simulink model "part1_pendulum_R2021a"  (R2021a)
settings: Solver=ode45  StartTime=0.0  StopTime=2  MaxStep=0.005  RelTol=1e-8  AbsTol=1e-10
model workspace (MAT data in the model file):
  g = 9.81
  k = 0.05
  l = 0.5
  m = 0.2
  omega0 = 0
  theta0 = 0.1
settings Model: Creator=matiasgarcia  LastModifiedBy=matiasgarcia
settings DataIOCC: SaveOutput=off  SignalLogging=off  SaveTime=off
settings DebuggingCC: UnconnectedInputMsg=none  UnconnectedOutputMsg=none  UnconnectedLineMsg=none
settings ModelReferenceCC: EnableRefExpFcnMdlSchedulingChecks=off
settings RTWCC: Description=Generic Real-Time Target  GPUComputeCapability=5.0  DLArmComputeVersion=20.02.1

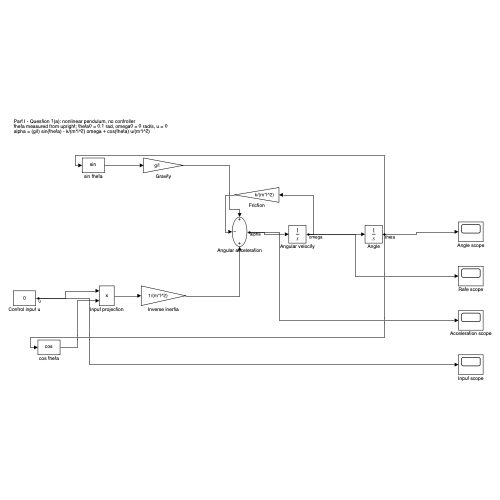
[thumbnail: Simulink's stored preview of the top-level diagram]
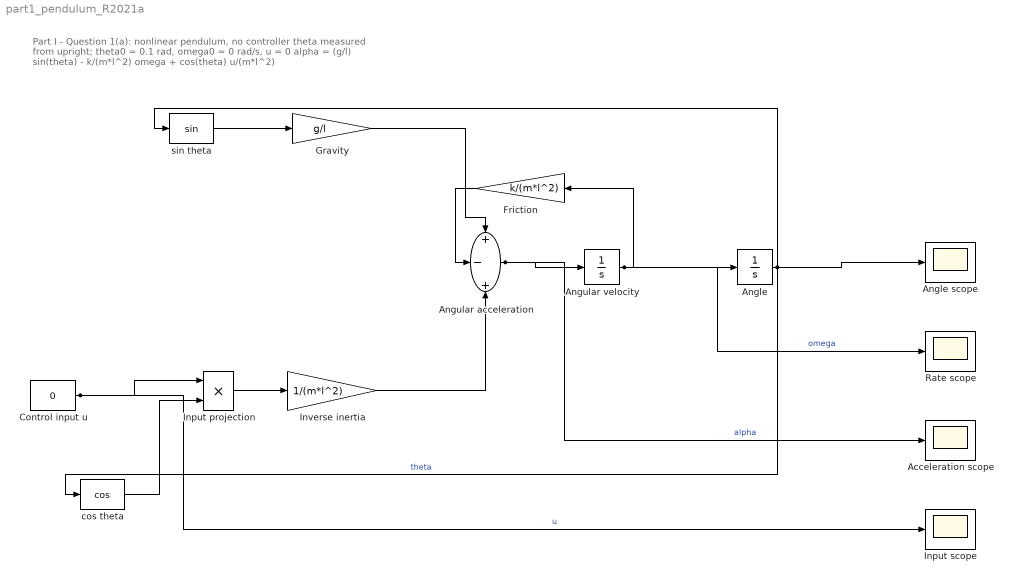
== system part1_pendulum_R2021a ==
  note: Part I - Question 1(a): nonlinear pendulum, no controller
      | theta measured from upright; theta0 = 0.1 rad, omega0 = 0 rad/s, u = 0
      | alpha = (g/l) sin(theta) - k/(m*l^2) omega + cos(theta) u/(m*l^2)
  Acceleration scope : Scope
  Angle : Integrator  InitialCondition=theta0
  Angle scope : Scope
  Angular acceleration : Sum  Inputs=+-+
  Angular velocity : Integrator  InitialCondition=omega0
  Control input u : Constant  Value=0
  Friction : Gain  Gain=k/(m*l^2)
  Gravity : Gain  Gain=g/l
  Input projection : Product
  Input scope : Scope
  Inverse inertia : Gain  Gain=1/(m*l^2)
  Rate scope : Scope
  cos theta : Trigonometry  Operator=cos
  sin theta : Trigonometry
  wires:
  Control input u/1 -> Input projection/1, Input scope/1  "u"
  cos theta/1 -> Input projection/2
  Input projection/1 -> Inverse inertia/1
  Inverse inertia/1 -> Angular acceleration/3
  sin theta/1 -> Gravity/1
  Gravity/1 -> Angular acceleration/1
  Angular velocity/1 -> Friction/1, Angle/1, Rate scope/1  "omega"
  Friction/1 -> Angular acceleration/2
  Angular acceleration/1 -> Angular velocity/1, Acceleration scope/1  "alpha"
  Angle/1 -> sin theta/1, cos theta/1, Angle scope/1  "theta"
